simulink model "sonobe2025_figure3"  (R2025b)
settings: Solver=ode45  StartTime=0.0  StopTime=40  MaxStep=0.005  RelTol=1e-3
model workspace (MAT data in the model file):
  Jb = 8
  Tv = 1
  g = 9.80665
  gamma_v = 0.02
  kd = 249.668888889
  kp = 662.22
  lb = 0.9
  mb = 60
  td = 0.155
  visual_sign = -1
settings Model: Creator=seguchi  LastModifiedBy=seguchi

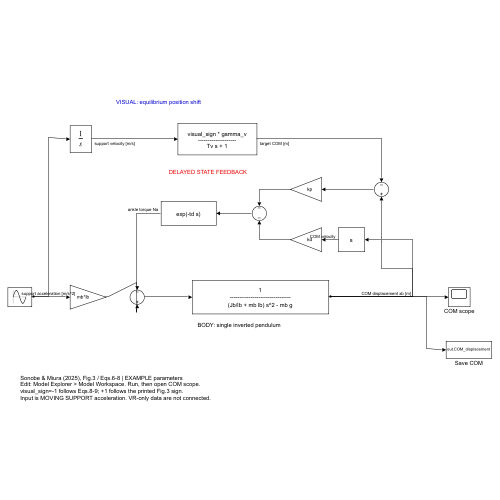
[thumbnail: Simulink's stored preview of the top-level diagram]
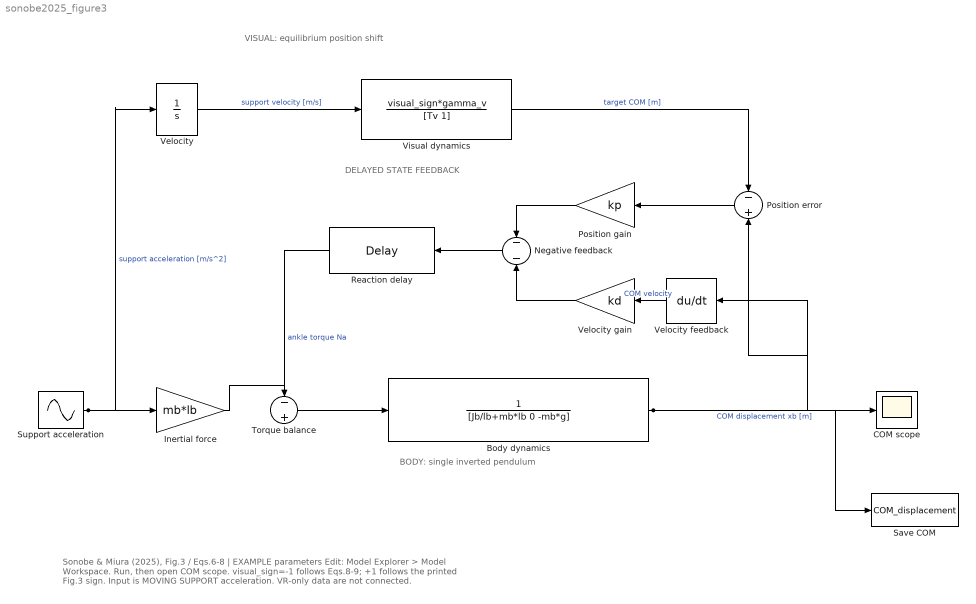
== system sonobe2025_figure3 ==
  note: VISUAL: equilibrium position shift
  note: DELAYED STATE FEEDBACK
  note: BODY: single inverted pendulum
  note: Sonobe & Miura (2025), Fig.3 / Eqs.6-8 | EXAMPLE parameters
      | Edit: Model Explorer > Model Workspace. Run, then open COM scope.
      | visual_sign=-1 follows Eqs.8-9; +1 follows the printed Fig.3 sign.
      | Input is MOVING SUPPORT acceleration. VR-only data are not connected.
  Body dynamics : TransferFcn  Numerator=1  Denominator=[Jb/lb+mb*lb 0 -mb*g]
      mask Display: text(0.5,0.73,'1','horizontalAlignment','center'); text(0.5,0.52,'--------------------------------','horizontalAlignment','center'); text(0.5,0.28,'(Jb/lb + mb lb) s^2 - mb g','horizontalAlignment','center');
  COM scope : Scope
  Inertial force : Gain  Gain=mb*lb
  Negative feedback : Sum  Inputs=--
  Position error : Sum  Inputs=-+
  Position gain : Gain  Gain=kp
  Reaction delay : TransportDelay  DelayTime=td
      mask Display: text(0.5,0.5,'exp(-td s)','horizontalAlignment','center');
  Save COM : ToWorkspace  VariableName=COM_displacement  SaveFormat=Timeseries  SampleTime=-1
  Support acceleration : Sin  Amplitude=0.02  Frequency=2*pi*0.2  SampleTime=0
  Torque balance : Sum  Inputs=-+
  Velocity : Integrator
  Velocity feedback : Derivative
      mask Display: text(0.5,0.5,'s','horizontalAlignment','center');
  Velocity gain : Gain  Gain=kd
  Visual dynamics : TransferFcn  Numerator=visual_sign*gamma_v  Denominator=[Tv 1]
      mask Display: text(0.5,0.68,'visual_sign * gamma_v','horizontalAlignment','center'); text(0.5,0.50,'--------------------','horizontalAlignment','center'); text(0.5,0.30,'Tv s + 1','horizontalAlignment','center');
  wires:
  Support acceleration/1 -> Inertial force/1, Velocity/1  "support acceleration [m/s^2]"
  Velocity/1 -> Visual dynamics/1  "support velocity [m/s]"
  Position error/1 -> Position gain/1
  Position gain/1 -> Negative feedback/1
  Velocity feedback/1 -> Velocity gain/1  "COM velocity"
  Velocity gain/1 -> Negative feedback/2
  Negative feedback/1 -> Reaction delay/1
  Reaction delay/1 -> Torque balance/2  "ankle torque Na"
  Inertial force/1 -> Torque balance/1
  Torque balance/1 -> Body dynamics/1
  Body dynamics/1 -> COM scope/1, Velocity feedback/1, Save COM/1, Position error/2  "COM displacement xb [m]"
  Visual dynamics/1 -> Position error/1  "target COM [m]"
